simulink model "E11"  (R2024a)
settings: Solver=VariableStepAuto  StartTime=0.0  StopTime=10.0  RelTol=1e-3
settings Model: Creator=Sanagostar  LastModifiedBy=Sanagostar

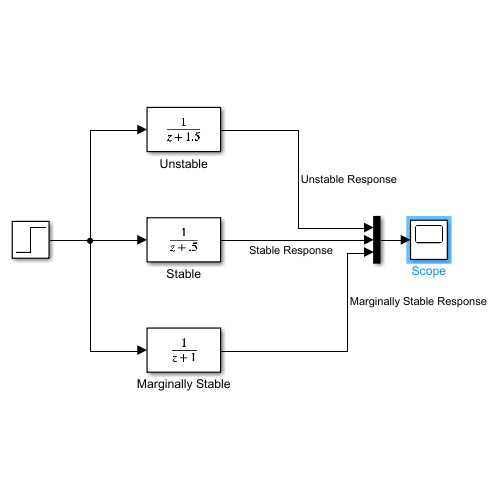
[thumbnail: Simulink's stored preview of the top-level diagram]
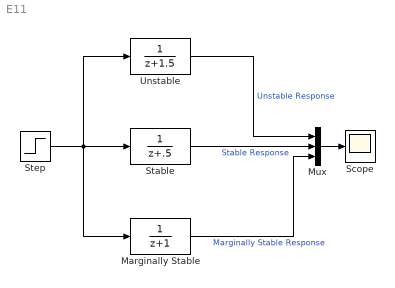
== system E11 ==
  Marginally Stable : DiscreteTransferFcn  Denominator=[1 1]
  Mux : Mux  Inputs=3
  Scope : Scope
  Stable : DiscreteTransferFcn  Denominator=[1 .5]
  Step : Step  SampleTime=0
  Unstable : DiscreteTransferFcn  Denominator=[1 1.5]
  wires:
  Unstable/1 -> Mux/1  "Unstable Response"
  Marginally Stable/1 -> Mux/3  "Marginally Stable Response"
  Step/1 -> Marginally Stable/1, Unstable/1, Stable/1
  Mux/1 -> Scope/1
  Stable/1 -> Mux/2  "Stable Response"
